simulink subsystem "Subsys_GFormConv_OuterCtrl_ZDepDroop"  (R2022b)
settings: Solver=VariableStepAuto  StartTime=0.0  StopTime=10.0  RelTol=1e-3
model mask{f_n=50, k_f=0.05, k_V=0.1, k_R=0, k_X=1, T_V=0.2, T_s_ctrl=1e-3, T_s_PWM_meas=1e-4}
  mask prompts: f_n "Nominal Frequency [Hz]"; k_f "Droop coefficient k_f (df/(dP+dQ))"; k_V "Droop coefficient k_V (dV/(dP+dQ))"; k_R "R/Z ratio"; k_X "X/Z ratio"; T_V "PT1 time constant voltage loop [s]"; T_s_ctrl "Controller sample time [s]"; T_s_PWM_meas "PWM and measurements sample time [s]"
undefined symbols (not defined in the file): alpha_LPF_V
libraries: simulink x1
settings Model: Creator=winkens  LastModifiedBy=winkens
settings SolverCC: AlgebraicLoopSolver=TrustRegion
settings DebuggingCC: UnconnectedInputMsg=warning  UnconnectedOutputMsg=warning  UnconnectedLineMsg=warning  SFMachineParentedDataDiag=warning
settings ModelReferenceCC: EnableRefExpFcnMdlSchedulingChecks=on
settings RTWCC: DLArmComputeVersion=19.05

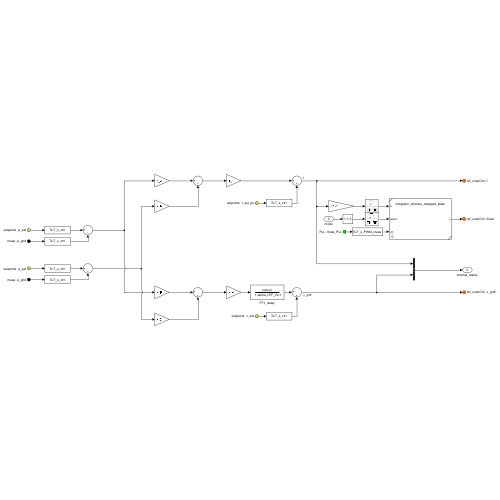
[thumbnail: Simulink's stored preview of the top-level diagram]
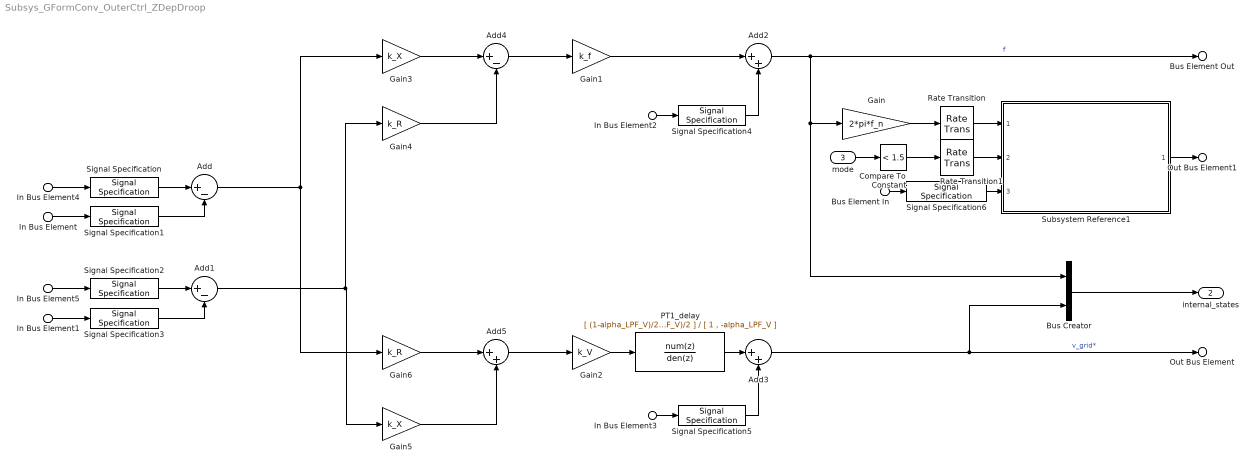
== system Subsys_GFormConv_OuterCtrl_ZDepDroop ==
  In Bus Element : Inport  PortName=meas  Element=p_grid
  In Bus Element1 : Inport  PortName=meas  Element=q_grid
  In Bus Element2 : Inport  Port=2  PortName=setpoints  Element=f_set_pu
  In Bus Element3 : Inport  Port=2  PortName=setpoints  Element=v_set
  In Bus Element4 : Inport  Port=2  PortName=setpoints  Element=p_set
  In Bus Element5 : Inport  Port=2  PortName=setpoints  Element=q_set
  mode : Inport  Port=3
  Bus Element In : Inport  Port=4  PortName=PLL  Element=theta_PLL
  Add : Sum  Inputs=|+-
  Add1 : Sum  Inputs=|+-
  Add2 : Sum  Inputs=|++
  Add3 : Sum  Inputs=|++
  Add4 : Sum  Inputs=|+-
  Add5 : Sum  Inputs=|++
  Bus Creator : BusCreator  Inputs=2
  Compare To Constant : simulink/Logic and Bit Operations/Compare To Constant  relop=<  const=1.5  OutDataTypeStr=boolean
  Gain : Gain  Gain=2*pi*f_n
  Gain1 : Gain  Gain=k_f
  Gain2 : Gain  Gain=k_V
  Gain3 : Gain  Gain=k_X
  Gain4 : Gain  Gain=k_R
  Gain5 : Gain  Gain=k_X
  Gain6 : Gain  Gain=k_R
  PT1_delay : DiscreteFilter  Numerator=[ (1-alpha_LPF_V)/2 , (1-alpha_LPF_V)/2 ]  Denominator=[ 1 , -alpha_LPF_V ]  SampleTime=T_s_ctrl
  Rate Transition : RateTransition  Deterministic=off  OutPortSampleTime=T_s_PWM_meas
  Rate Transition1 : RateTransition  Deterministic=off  OutPortSampleTime=T_s_PWM_meas
  Signal Specification{,1..5} (6 alike) : SignalSpecification  SampleTime=T_s_ctrl
  Signal Specification6 : SignalSpecification  SampleTime=T_s_PWM_meas
  Subsystem Reference1 : Subsystem  ReferencedSubsystem=Integrator_discrete_wrapped_state  WrappedStateUpperValue=2*pi  WrappedStateLowerValue=0  x_0=0  T_s=T_s_PWM_meas
  Out Bus Element1 : Outport  PortName=ref_outerCtrl  Element=theta
  Bus Element Out : Outport  PortName=ref_outerCtrl  Element=f
  Out Bus Element : Outport  PortName=ref_outerCtrl  Element=v_grid*
  internal_states : Outport  Port=2
  wires:
  Subsystem Reference1/1 -> Out Bus Element1/1
  Gain/1 -> Rate Transition/1
  mode/1 -> Compare To Constant/1
  Compare To Constant/1 -> Rate Transition1/1
  Bus Element In/1 -> Signal Specification6/1
  Bus Creator/1 -> internal_states/1
  Add3/1 -> Bus Creator/2, Out Bus Element/1  "v_grid*"
  Add2/1 -> Bus Element Out/1, Gain/1, Bus Creator/1  "f"
  In Bus Element4/1 -> Signal Specification/1
  In Bus Element5/1 -> Signal Specification2/1
  In Bus Element/1 -> Signal Specification1/1
  In Bus Element1/1 -> Signal Specification3/1
  In Bus Element3/1 -> Signal Specification5/1
  In Bus Element2/1 -> Signal Specification4/1
  Gain1/1 -> Add2/1
  Gain2/1 -> PT1_delay/1
  Add4/1 -> Gain1/1
  Add5/1 -> Gain2/1
  Gain3/1 -> Add4/1
  Gain4/1 -> Add4/2
  Gain6/1 -> Add5/1
  Gain5/1 -> Add5/2
  Add/1 -> Gain6/1, Gain3/1
  Add1/1 -> Gain4/1, Gain5/1
  PT1_delay/1 -> Add3/1
  Signal Specification/1 -> Add/1
  Signal Specification1/1 -> Add/2
  Signal Specification2/1 -> Add1/1
  Signal Specification3/1 -> Add1/2
  Signal Specification4/1 -> Add2/2
  Signal Specification5/1 -> Add3/2
  Signal Specification6/1 -> Subsystem Reference1/3
  Rate Transition1/1 -> Subsystem Reference1/2
  Rate Transition/1 -> Subsystem Reference1/1
